simulink model "HW1_Benchmark"  (R2023b)
settings: Solver=VariableStepAuto  StartTime=0.0  StopTime=1000  RelTol=1e-3
libraries: dspxfrm3 x2, commdigbbndam3 x2, commchan3 x1, commsink2 x1, commrandsrc3 x1
settings Model: Creator=Vibha  LastModifiedBy=chang
settings SolverCC: AlgebraicLoopSolver=TrustRegion
settings DataIOCC: ReturnWorkspaceOutputs=off
settings DebuggingCC: UnconnectedInputMsg=warning  UnconnectedOutputMsg=warning  UnconnectedLineMsg=warning  ArithmeticOperatorsInVariantConditions=warning
settings ModelReferenceCC: EnableRefExpFcnMdlSchedulingChecks=on
settings SFSimCC: SimUseLocalCustomCode=off  CustomCodeUndefinedFunction=UseInterfaceOnly
settings RTWCC: RTWUseLocalCustomCode=off
settings CodeAppCC: StateflowObjectComments=on

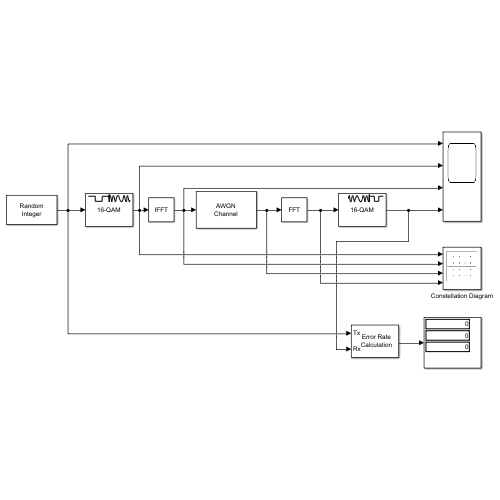
[thumbnail: Simulink's stored preview of the top-level diagram]
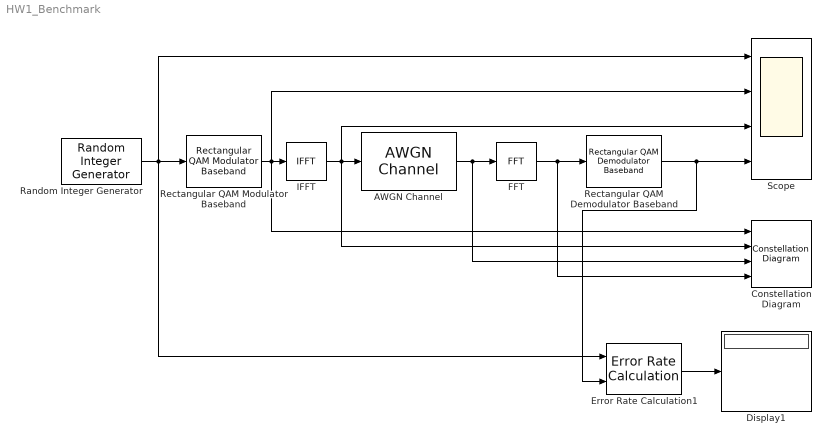
== system HW1_Benchmark ==
  AWGN Channel : commchan3/AWGN Channel  LegacyMode=on  NoiseMethod="Signal to noise ratio  (SNR)"  noiseMode="Signal to noise ratio  (Eb/No)"  EbNo=40  EsNo=10  SNR=10  BitsPerSymbol=2  SignalPower=1  SamplesPerSymbol=1  SymbolPeriod=1  VarianceSource=Parameter  Variance=1  RandomStream=Global stream  Seed=67  SimulateUsing=Code generation
  Constellation Diagram : ConstellationDiagram  NumInputPorts=4  WindowPosition=[1419.000000,154.000000,600.000000,600.000000,]  Visible=on  ScopeFrameLocation=window  ReferenceConstellation="{[0.7071+0.7071i          -0.7071+0.7071i          -0.7071-0.7071i            0.707-0.7071i][0.7071+0.7071i          -0.7071+0.7071i          -0.7071-0.7071i            0.707-0.7071i][0.7071+0.7071i          -0.7071+0.7071i          -0.7071-0.7071i            0.707-0.7071i][0.7071+0.7071i          -0.7071+0.7071i          -0.7071-0.7071i            0.707-0.7071i]}"  ShowLegend=on
  Display1 : Display
  Error Rate Calculation1 : commsink2/Error Rate Calculation  N=0  st_delay=0  cp_mode=Entire frame  subframe=[]  PMode=Port  WsName=ErrorVec  RsMode2=off  stop=off  numErr=100  maxBits=1e6
  FFT : dspxfrm3/FFT  FFTImplementation=Auto  CompMethod=Table lookup  TableOpt=NEW  TableOptActive=Speed  BitRevOrder=off  Normalize=off  InheritFFTLength=on  FFTLength=64  WrapInput=on  roundingMode=Floor  overflowMode=off  firstCoeffDataTypeStr=Inherit: Same word length as input  firstCoeffLastDataTypeStr=Inherit: Same word length as input  outputMin=[]  outputMax=[]
  IFFT : dspxfrm3/IFFT  FFTImplementation=Auto  CompMethod=Table lookup  TableOpt=NEW  TableOptActive=Speed  BitRevOrder=off  cs_in=off  Normalize=on  InheritFFTLength=on  FFTLength=64  WrapInput=on  mode=Complex  outSamplingMode=Sample based  roundingMode=Floor  overflowMode=off  firstCoeffDataTypeStr=Inherit: Same word length as input  firstCoeffLastDataTypeStr=Inherit: Same word length as input  outputMin=[]  outputMax=[]
  Random Integer Generator : commrandsrc3/Random Integer Generator  SetSize=16  SeedSource=Parameter  Seed=37  SampleTime=1  SamplesPerFrame=128  OutputDataType=double  SimulateUsing=Interpreted execution
  Rectangular QAM Demodulator Baseband : commdigbbndam3/Rectangular QAM Demodulator Baseband  M=16  OutType=Integer  DecType=Hard decision  VarSource=Dialog  Variance=1  Dec=Gray  Mapping=[0:15]  PowType=Average Power  MinDist=2  AvgPow=1  PeakPow=1  Ph=0  outDtype1=Inherit via internal rule  outDtype2=Inherit via internal rule  derotateFactorWordLen=16  derotateFactorDataTypeStr=Inherit: Same word length as input  derotateFactorLastDataTypeStr=Inherit: Same word length as input  denormFactorWordLen=16  denormFactorDataTypeStr=Inherit: Same word length as input  denormFactorLastDataTypeStr=Inherit: Same word length as input  prodOutWordLen=32  prodOutOverflowMode=Wrap  prodOutRoundingMode=Floor  prodOutOvFlMode=off  prodOutOvFlModeLastStrValue=off  sumWordLen=32
  Rectangular QAM Modulator Baseband : commdigbbndam3/Rectangular QAM Modulator Baseband  M=16  InType=Integer  Enc=Gray  Mapping=[0:15]  PowType=Average Power  MinDist=2  AvgPow=1  PeakPow=1  Ph=0  outDtype=double  outWordLen=16  outUDDataType=sfix(16)  outFracLenMode=Best precision  outFracLen=15  outDataTypeStr=double  outLastDataTypeStr=double
  Scope : Scope  NumInputPorts=4
  wires:
  Rectangular QAM Demodulator Baseband/1 -> Error Rate Calculation1/2, Scope/4
  Random Integer Generator/1 -> Error Rate Calculation1/1, Scope/1, Rectangular QAM Modulator Baseband/1
  Rectangular QAM Modulator Baseband/1 -> Scope/2, Constellation Diagram/1, IFFT/1
  IFFT/1 -> Constellation Diagram/2, Scope/3, AWGN Channel/1
  AWGN Channel/1 -> Constellation Diagram/3, FFT/1
  FFT/1 -> Constellation Diagram/4, Rectangular QAM Demodulator Baseband/1
  Error Rate Calculation1/1 -> Display1/1
